simulink model "clutch_debug_simulink"  (R2024b)
settings: Solver=ode15s  StartTime=0.0  StopTime=4  MaxStep=0.002  RelTol=1e-6  AbsTol=1e-8
model workspace (MAT data in the model file):
  J_input = 0.00354192570756
  J_load = 2000
  M_debug = 100
  N_clutch = 230
  clutch1_profile = [0  0; 0.05  0; 0.06  0.1; 0.5  0.1; 0.7  1; 3  1; 3.1  0; 4  0]
  clutch2_profile = [0  0; 4  0]
  mi_c = 0.3
  mi_s = 0.4
  n_surfaces = 20
  r_eq_clutch = 0.1
  ratio1 = 3
  ratio2 = 1.5
  sigma0 = 335063
  sigma1 = 10
  sigma2 = 0
  vs = 0.5
libraries: simulink x6
settings Model: Creator=menda  LastModifiedBy=menda

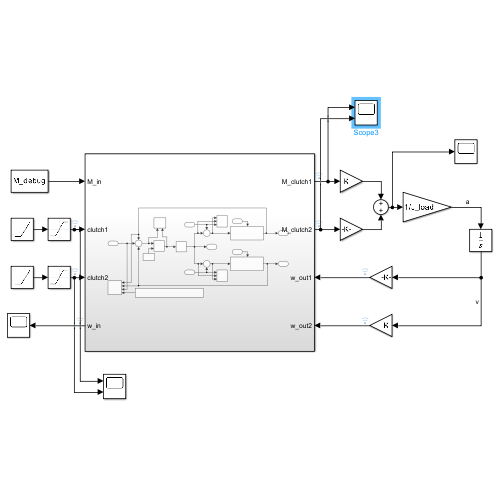
[thumbnail: Simulink's stored preview of the top-level diagram]
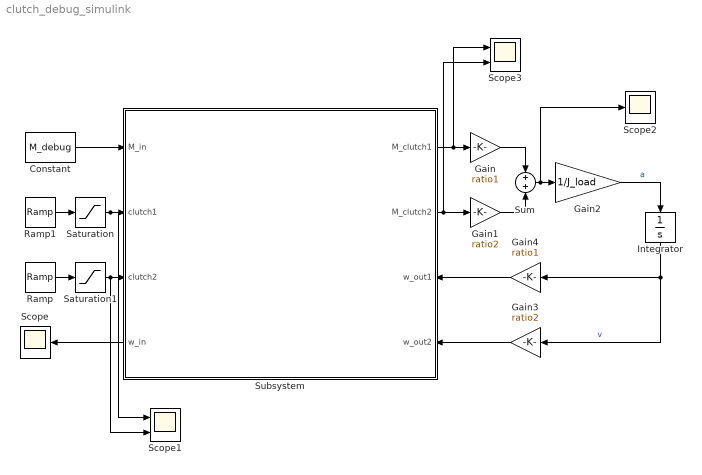
== system clutch_debug_simulink ==
  Constant : Constant  Value=M_debug
  Gain : Gain  Gain=ratio1
  Gain1 : Gain  Gain=ratio2
  Gain2 : Gain  Gain=1/J_load
  Gain3 : Gain  Gain=ratio2
  Gain4 : Gain  Gain=ratio1
  Integrator : Integrator  InitialCondition=100
  Ramp : simulink/Sources/Ramp  slope=3  start=1  InitialOutput=0
  Ramp1 : simulink/Sources/Ramp  slope=-3  start=1  InitialOutput=1
  Saturation : Saturate  UpperLimit=1  LowerLimit=0
  Saturation1 : Saturate  UpperLimit=1  LowerLimit=0
  Scope : Scope
  Scope1 : Scope  NumInputPorts=2
  Scope2 : Scope
  Scope3 : Scope  NumInputPorts=2
  Subsystem : Subsystem
      settings: PortSchema="{\"entries\":[{\"content\":{\"sides\":[{\"content\":{\"connectorIds\":[\"In1\",\"In2\",\"In3\",\"Out3\"]},\"type\":\"ConnectorPlacement.EquallySpacedRectSide\",\"uuid\":\"80fb4076-f99e-49a2-a4a4-074ad4e3703f\"},{\"content\":{\"connectorIds\":[\"Out1\",\"Out2\",\"In4\",\"In5\"],\"side\":\"RIGHT\"},\"type\":\"ConnectorPlacement.EquallySpacedRectSide\",\"uuid\":\"6fd981d1-b0c4-4e88-a9ee-be732220d23b\"},{\"content\":{\"side\":\"TOP\"},\"type\":\"ConnectorPlacement.EquallySpacedRectSide\",\"uuid\":\"d51b7d36-7666-4ef4-83a7-fb6ef995ec7f\"}]},\"type\":\"ConnectorPlacement.EquallySpacedConnector\",\"uuid\":\"9caa9749-ac4c-4898-95ff-5d55f9fdcdc9\"}],\"packageUris\":[\"http://schema.mathworks.com/mf0/Connector/R2020b\"],\"version\":\"1.0\"}"
  Sum : Sum  Inputs=+|+
  wires:
  Subsystem/1(M_clutch1) -> Scope3/1, Gain/1
  Subsystem/2(M_clutch2) -> Gain1/1, Scope3/2
  Constant/1 -> Subsystem/1(M_in)
  Saturation/1 -> Scope1/1, Subsystem/2(clutch1)
  Saturation1/1 -> Scope1/2, Subsystem/3(clutch2)
  Subsystem/3(w_in) -> Scope/1
  Gain/1 -> Sum/1
  Gain1/1 -> Sum/2
  Sum/1 -> Scope2/1, Gain2/1
  Gain2/1 -> Integrator/1  "a"
  Integrator/1 -> Gain3/1, Gain4/1  "v"
  Gain3/1 -> Subsystem/5(w_out2)
  Gain4/1 -> Subsystem/4(w_out1)
  Ramp1/1 -> Saturation/1
  Ramp/1 -> Saturation1/1

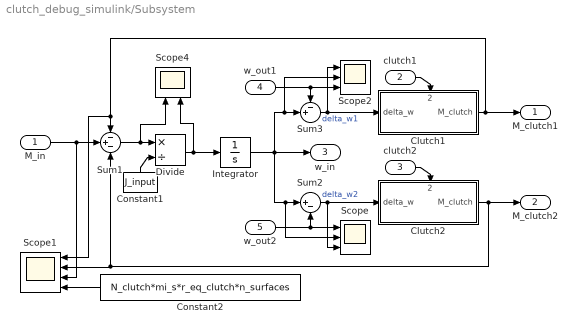
== system clutch_debug_simulink/Subsystem ==
  M_in : Inport
  clutch1 : Inport  Port=2
  clutch2 : Inport  Port=3
  w_out1 : Inport  Port=4
  w_out2 : Inport  Port=5
  Clutch1 : Subsystem
      settings: PortSchema="{\"entries\":[{\"content\":{\"sides\":[{\"content\":{\"connectorIds\":[\"In1\"]},\"type\":\"ConnectorPlacement.EquallySpacedRectSide\",\"uuid\":\"a26f5a32-9f9c-4306-b7a8-6355090a4a86\"},{\"content\":{\"connectorIds\":[\"Out1\"],\"side\":\"RIGHT\"},\"type\":\"ConnectorPlacement.EquallySpacedRectSide\",\"uuid\":\"4fa489e2-cd1d-4a36-b0cb-261100046200\"},{\"content\":{\"connectorIds\":[\"In2\"],\"side\":\"TOP\"},\"type\":\"ConnectorPlacement.EquallySpacedRectSide\",\"uuid\":\"0e05a540-d6e3-4351-9a32-83f6c32571ff\"}]},\"type\":\"ConnectorPlacement.EquallySpacedConnector\",\"uuid\":\"492e0439-728a-4999-b29b-e2639b0e762e\"}],\"packageUris\":[\"http://schema.mathworks.com/mf0/Connector/R2020b\"],\"version\":\"1.0\"}"
  Clutch2 : Subsystem
      settings: PortSchema="{\"entries\":[{\"content\":{\"sides\":[{\"content\":{\"connectorIds\":[\"In1\"]},\"type\":\"ConnectorPlacement.EquallySpacedRectSide\",\"uuid\":\"a26f5a32-9f9c-4306-b7a8-6355090a4a86\"},{\"content\":{\"connectorIds\":[\"Out1\"],\"side\":\"RIGHT\"},\"type\":\"ConnectorPlacement.EquallySpacedRectSide\",\"uuid\":\"4fa489e2-cd1d-4a36-b0cb-261100046200\"},{\"content\":{\"connectorIds\":[\"In2\"],\"side\":\"TOP\"},\"type\":\"ConnectorPlacement.EquallySpacedRectSide\",\"uuid\":\"0e05a540-d6e3-4351-9a32-83f6c32571ff\"}]},\"type\":\"ConnectorPlacement.EquallySpacedConnector\",\"uuid\":\"492e0439-728a-4999-b29b-e2639b0e762e\"}],\"packageUris\":[\"http://schema.mathworks.com/mf0/Connector/R2020b\"],\"version\":\"1.0\"}"
  Constant1 : Constant  Value=J_input
  Constant2 : Constant  Value=N_clutch*mi_s*r_eq_clutch*n_surfaces
  Divide : Product  Inputs=*/
  Integrator : Integrator  InitialCondition=100
  Scope : Scope  NumInputPorts=3
  Scope1 : Scope  NumInputPorts=4
  Scope2 : Scope  NumInputPorts=3
  Scope4 : Scope  NumInputPorts=2
  Sum1 : Sum  Inputs=-+-
  Sum2 : Sum  Inputs=|+-
  Sum3 : Sum  Inputs=-+|
  M_clutch1 : Outport
  M_clutch2 : Outport  Port=2
  w_in : Outport  Port=3
  wires:
  Sum3/1 -> Clutch1/1(delta_w), Scope2/1  "delta_w1"
  w_out1/1 -> Scope2/3, Sum3/1
  Clutch2/1(M_clutch) -> M_clutch2/1, Scope1/2, Sum1/3
  Sum1/1 -> Scope4/1, Divide/1
  Constant1/1 -> Divide/2
  w_out2/1 -> Scope/1, Sum2/2
  Integrator/1 -> w_in/1, Scope/2, Sum2/1, Scope2/2, Sum3/2
  Clutch1/1(M_clutch) -> M_clutch1/1, Scope1/1, Sum1/1
  clutch1/1 -> Clutch1/2(" ")
  Divide/1 -> Integrator/1, Scope4/2
  Constant2/1 -> Scope1/4
  Sum2/1 -> Clutch2/1(delta_w), Scope/3  "delta_w2"
  M_in/1 -> Sum1/2, Scope1/3
  clutch2/1 -> Clutch2/2(" ")

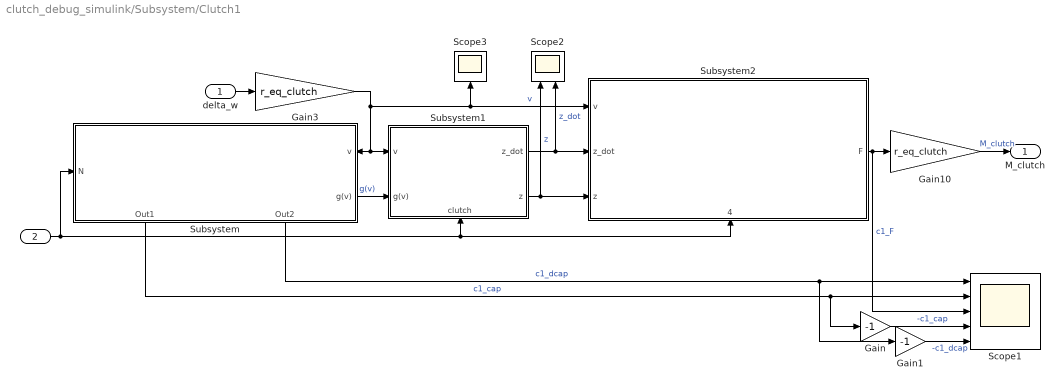
== system clutch_debug_simulink/Subsystem/Clutch1 ==
  delta_w : Inport
  " " : Inport  Port=2
  Gain : Gain  Gain=-1
  Gain1 : Gain  Gain=-1
  Gain10 : Gain  Gain=r_eq_clutch
  Gain3 : Gain  Gain=r_eq_clutch
  Scope1 : Scope  NumInputPorts=5
  Scope2 : Scope  NumInputPorts=2
  Scope3 : Scope
  Subsystem : Subsystem
      settings: PortSchema="{\"entries\":[{\"content\":{\"sides\":[{\"content\":{\"connectorIds\":[\"In1\"]},\"type\":\"ConnectorPlacement.EquallySpacedRectSide\",\"uuid\":\"0ae2ed28-5be6-4ce0-b87c-2c13a72d1ad0\"},{\"content\":{\"connectorIds\":[\"In2\",\"Out1\"],\"side\":\"RIGHT\"},\"type\":\"ConnectorPlacement.EquallySpacedRectSide\",\"uuid\":\"8d48d664-ebaf-4c3e-be9e-f793543e8061\"},{\"content\":{\"side\":\"TOP\"},\"type\":\"ConnectorPlacement.EquallySpacedRectSide\",\"uuid\":\"2d66836a-de46-4974-a48b-ee2778be1c08\"},{\"content\":{\"connectorIds\":[\"Out2\",\"Out3\"],\"side\":\"BOTTOM\"},\"type\":\"ConnectorPlacement.EquallySpacedRectSide\",\"uuid\":\"e232d9f4-6257-4976-8384-26c462ae0041\"}]},\"type\":\"ConnectorPlacement.EquallySpacedConnector\",\"uuid\":\"ae24f926-3a59-4a74-9cf0-af55dcfbad19\"}],\"packageUris\":[\"http://schema.mathworks.com/mf0/Connector/R2020b\"],\"version\":\"1.0\"}"
      mask Display: image('images/Stribeck.png');
  Subsystem1 : Subsystem
      settings: PortSchema="{\"entries\":[{\"content\":{\"sides\":[{\"content\":{\"connectorIds\":[\"In1\",\"In2\"]},\"type\":\"ConnectorPlacement.EquallySpacedRectSide\",\"uuid\":\"fba00446-fe01-4fd0-a740-7d5efbf0abc7\"},{\"content\":{\"connectorIds\":[\"Out1\",\"Out2\"],\"side\":\"RIGHT\"},\"type\":\"ConnectorPlacement.EquallySpacedRectSide\",\"uuid\":\"28d31996-59d3-4656-988b-c785e0d07c46\"},{\"content\":{\"side\":\"TOP\"},\"type\":\"ConnectorPlacement.EquallySpacedRectSide\",\"uuid\":\"07dfb693-bdac-419f-bf8c-22f11bb5a1ff\"},{\"content\":{\"connectorIds\":[\"In3\"],\"side\":\"BOTTOM\"},\"type\":\"ConnectorPlacement.EquallySpacedRectSide\",\"uuid\":\"e46b7f0d-22dc-4b01-9fc3-2183fe5bd14e\"}]},\"type\":\"ConnectorPlacement.EquallySpacedConnector\",\"uuid\":\"53afe5e8-6f41-4676-b5a4-a094561728b0\"}],\"packageUris\":[\"http://schema.mathworks.com/mf0/Connector/R2020b\"],\"version\":\"1.0\"}"
      mask Display: image('images/z_state.png');
  Subsystem2 : Subsystem
      settings: PortSchema="{\"entries\":[{\"content\":{\"sides\":[{\"content\":{\"connectorIds\":[\"In1\",\"In2\",\"In3\"]},\"type\":\"ConnectorPlacement.EquallySpacedRectSide\",\"uuid\":\"718e9a4c-012a-432e-af1d-56a8c510a1ff\"},{\"content\":{\"connectorIds\":[\"Out1\"],\"side\":\"RIGHT\"},\"type\":\"ConnectorPlacement.EquallySpacedRectSide\",\"uuid\":\"b8acef94-ef29-40e0-b6df-913e21cb4db2\"},{\"content\":{\"side\":\"TOP\"},\"type\":\"ConnectorPlacement.EquallySpacedRectSide\",\"uuid\":\"42ba6916-bf07-457b-89e7-b10a87e70d96\"},{\"content\":{\"connectorIds\":[\"In4\"],\"side\":\"BOTTOM\"},\"type\":\"ConnectorPlacement.EquallySpacedRectSide\",\"uuid\":\"25c3a005-357f-4967-9fb3-686ba180841f\"}]},\"type\":\"ConnectorPlacement.EquallySpacedConnector\",\"uuid\":\"db3b50fc-f4cd-400b-b8f7-b0301a8ba65b\"}],\"packageUris\":[\"http://schema.mathworks.com/mf0/Connector/R2020b\"],\"version\":\"1.0\"}"
      mask Display: image('images/fric_force.png');
  M_clutch : Outport
  wires:
  delta_w/1 -> Gain3/1
  Subsystem1/2(z) -> Scope2/1, Subsystem2/3(z)  "z"
  Subsystem1/1(z_dot) -> Scope2/2, Subsystem2/2(z_dot)  "z_dot"
  Subsystem2/1(F) -> Scope1/3, Gain10/1  "c1_F"
  Gain10/1 -> M_clutch/1  "M_clutch"
  Gain3/1 -> Scope3/1, Subsystem2/1(v), Subsystem1/1(v), Subsystem/2(v)  "v"
  Subsystem/1(g(v)) -> Subsystem1/2(g(v))  "g(v)"
  " "/1 -> Subsystem2/4(" "), Subsystem1/3("clutch "), Subsystem/1(N)
  Subsystem/2(Out1) -> Gain/1, Scope1/2  "c1_cap"
  Gain/1 -> Scope1/4  "-c1_cap"
  Subsystem/3(Out2) -> Gain1/1, Scope1/1  "c1_dcap"
  Gain1/1 -> Scope1/5  "-c1_dcap"

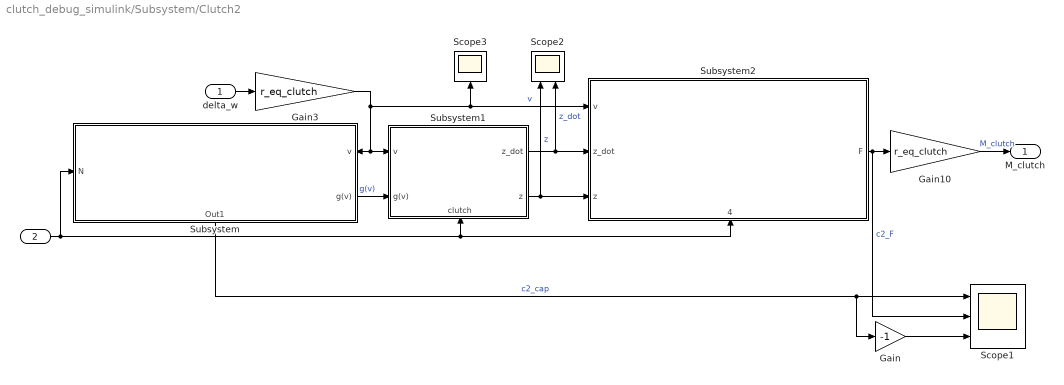
== system clutch_debug_simulink/Subsystem/Clutch2 ==
  delta_w : Inport
  " " : Inport  Port=2
  Gain : Gain  Gain=-1
  Gain10 : Gain  Gain=r_eq_clutch
  Gain3 : Gain  Gain=r_eq_clutch
  Scope1 : Scope  NumInputPorts=3
  Scope2 : Scope  NumInputPorts=2
  Scope3 : Scope
  Subsystem : Subsystem
      settings: PortSchema="{\"entries\":[{\"content\":{\"sides\":[{\"content\":{\"connectorIds\":[\"In1\"]},\"type\":\"ConnectorPlacement.EquallySpacedRectSide\",\"uuid\":\"0ae2ed28-5be6-4ce0-b87c-2c13a72d1ad0\"},{\"content\":{\"connectorIds\":[\"In2\",\"Out1\"],\"side\":\"RIGHT\"},\"type\":\"ConnectorPlacement.EquallySpacedRectSide\",\"uuid\":\"8d48d664-ebaf-4c3e-be9e-f793543e8061\"},{\"content\":{\"side\":\"TOP\"},\"type\":\"ConnectorPlacement.EquallySpacedRectSide\",\"uuid\":\"2d66836a-de46-4974-a48b-ee2778be1c08\"},{\"content\":{\"connectorIds\":[\"Out2\"],\"side\":\"BOTTOM\"},\"type\":\"ConnectorPlacement.EquallySpacedRectSide\",\"uuid\":\"e232d9f4-6257-4976-8384-26c462ae0041\"}]},\"type\":\"ConnectorPlacement.EquallySpacedConnector\",\"uuid\":\"ae24f926-3a59-4a74-9cf0-af55dcfbad19\"}],\"packageUris\":[\"http://schema.mathworks.com/mf0/Connector/R2020b\"],\"version\":\"1.0\"}"
      mask Display: image('images/Stribeck.png');
  Subsystem1 : Subsystem
      settings: PortSchema="{\"entries\":[{\"content\":{\"sides\":[{\"content\":{\"connectorIds\":[\"In1\",\"In2\"]},\"type\":\"ConnectorPlacement.EquallySpacedRectSide\",\"uuid\":\"fba00446-fe01-4fd0-a740-7d5efbf0abc7\"},{\"content\":{\"connectorIds\":[\"Out1\",\"Out2\"],\"side\":\"RIGHT\"},\"type\":\"ConnectorPlacement.EquallySpacedRectSide\",\"uuid\":\"28d31996-59d3-4656-988b-c785e0d07c46\"},{\"content\":{\"side\":\"TOP\"},\"type\":\"ConnectorPlacement.EquallySpacedRectSide\",\"uuid\":\"07dfb693-bdac-419f-bf8c-22f11bb5a1ff\"},{\"content\":{\"connectorIds\":[\"In3\"],\"side\":\"BOTTOM\"},\"type\":\"ConnectorPlacement.EquallySpacedRectSide\",\"uuid\":\"e46b7f0d-22dc-4b01-9fc3-2183fe5bd14e\"}]},\"type\":\"ConnectorPlacement.EquallySpacedConnector\",\"uuid\":\"53afe5e8-6f41-4676-b5a4-a094561728b0\"}],\"packageUris\":[\"http://schema.mathworks.com/mf0/Connector/R2020b\"],\"version\":\"1.0\"}"
      mask Display: image('images/z_state.png');
  Subsystem2 : Subsystem
      settings: PortSchema="{\"entries\":[{\"content\":{\"sides\":[{\"content\":{\"connectorIds\":[\"In1\",\"In2\",\"In3\"]},\"type\":\"ConnectorPlacement.EquallySpacedRectSide\",\"uuid\":\"718e9a4c-012a-432e-af1d-56a8c510a1ff\"},{\"content\":{\"connectorIds\":[\"Out1\"],\"side\":\"RIGHT\"},\"type\":\"ConnectorPlacement.EquallySpacedRectSide\",\"uuid\":\"b8acef94-ef29-40e0-b6df-913e21cb4db2\"},{\"content\":{\"side\":\"TOP\"},\"type\":\"ConnectorPlacement.EquallySpacedRectSide\",\"uuid\":\"42ba6916-bf07-457b-89e7-b10a87e70d96\"},{\"content\":{\"connectorIds\":[\"In4\"],\"side\":\"BOTTOM\"},\"type\":\"ConnectorPlacement.EquallySpacedRectSide\",\"uuid\":\"25c3a005-357f-4967-9fb3-686ba180841f\"}]},\"type\":\"ConnectorPlacement.EquallySpacedConnector\",\"uuid\":\"db3b50fc-f4cd-400b-b8f7-b0301a8ba65b\"}],\"packageUris\":[\"http://schema.mathworks.com/mf0/Connector/R2020b\"],\"version\":\"1.0\"}"
      mask Display: image('images/fric_force.png');
  M_clutch : Outport
  wires:
  Subsystem/2(Out1) -> Gain/1, Scope1/1  "c2_cap"
  " "/1 -> Subsystem/1(N), Subsystem1/3("clutch "), Subsystem2/4(" ")
  Subsystem/1(g(v)) -> Subsystem1/2(g(v))  "g(v)"
  Gain3/1 -> Subsystem/2(v), Subsystem1/1(v), Subsystem2/1(v), Scope3/1  "v"
  Gain10/1 -> M_clutch/1  "M_clutch"
  Subsystem2/1(F) -> Gain10/1, Scope1/2  "c2_F"
  Subsystem1/1(z_dot) -> Subsystem2/2(z_dot), Scope2/2  "z_dot"
  Subsystem1/2(z) -> Subsystem2/3(z), Scope2/1  "z"
  delta_w/1 -> Gain3/1
  Gain/1 -> Scope1/3

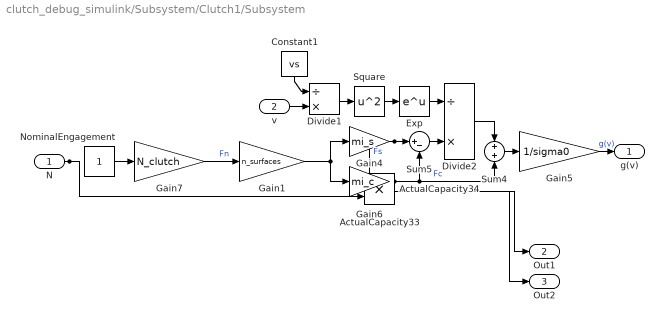
== system clutch_debug_simulink/Subsystem/Clutch1/Subsystem ==
  N : Inport
  v : Inport  Port=2
  ActualCapacity33 : Product
  ActualCapacity34 : Product
  Constant1 : Constant  Value=vs
  Divide1 : Product  Inputs=/*
  Divide2 : Product  Inputs=/*
  Exp : Math
  Gain1 : Gain  Gain=n_surfaces
  Gain4 : Gain  Gain=mi_s
  Gain5 : Gain  Gain=1/sigma0
  Gain6 : Gain  Gain=mi_c
  Gain7 : Gain  Gain=N_clutch
  NominalEngagement : Constant
  Square : Math  Operator=square
  Sum4 : Sum  Inputs=+|+
  Sum5 : Sum  Inputs=|+-
  g(v) : Outport
  Out1 : Outport  Port=2
  Out2 : Outport  Port=3
  wires:
  Gain1/1 -> Gain4/1, Gain6/1
  Gain4/1 -> Sum5/1, ActualCapacity33/1  "Fs"
  v/1 -> Divide1/2
  N/1 -> ActualCapacity33/2, ActualCapacity34/2
  Gain5/1 -> g(v)/1  "g(v)"
  Square/1 -> Exp/1
  Divide1/1 -> Square/1
  Constant1/1 -> Divide1/1
  Gain7/1 -> Gain1/1  "Fn"
  Exp/1 -> Divide2/1
  Gain6/1 -> Sum5/2, Sum4/2, ActualCapacity34/1  "Fc"
  Divide2/1 -> Sum4/1
  Sum5/1 -> Divide2/2
  Sum4/1 -> Gain5/1
  NominalEngagement/1 -> Gain7/1
  ActualCapacity33/1 -> Out1/1
  ActualCapacity34/1 -> Out2/1

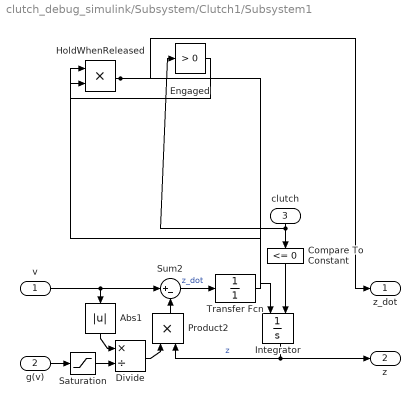
== system clutch_debug_simulink/Subsystem/Clutch1/Subsystem1 ==
  v : Inport
  g(v) : Inport  Port=2
  "clutch " : Inport  Port=3
  Abs1 : Abs  SaturateOnIntegerOverflow=off
  Compare To Constant : simulink/Logic and Bit Operations/Compare To Constant  relop=<=  const=0  OutDataTypeStr=boolean
  Divide : Product  Inputs=*/
  Engaged : simulink/Logic and Bit Operations/Compare To Constant  relop=>  const=0  OutDataTypeStr=boolean
  HoldWhenReleased : Product
  Integrator : Integrator  ExternalReset=rising
  Product2 : Product
  Saturation : Saturate  UpperLimit=inf  LowerLimit=1e-12
  Sum2 : Sum  Inputs=|+-
  Transfer Fcn : TransferFcn  Numerator=1  Denominator=1
  z_dot : Outport
  z : Outport  Port=2
  wires:
  Compare To Constant/1 -> Integrator/2
  g(v)/1 -> Saturation/1
  Product2/1 -> Sum2/2
  Abs1/1 -> Divide/1
  Saturation/1 -> Divide/2
  Sum2/1 -> Transfer Fcn/1  "z_dot"
  v/1 -> Sum2/1, Abs1/1
  Divide/1 -> Product2/1
  Integrator/1 -> z/1, Product2/2  "z"
  "clutch "/1 -> Compare To Constant/1, Engaged/1
  Transfer Fcn/1 -> HoldWhenReleased/1
  Engaged/1 -> HoldWhenReleased/2
  HoldWhenReleased/1 -> z_dot/1, Integrator/1

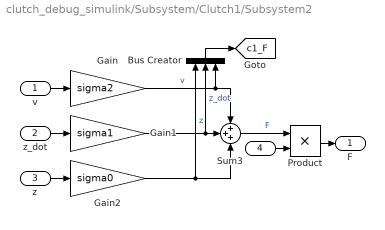
== system clutch_debug_simulink/Subsystem/Clutch1/Subsystem2 ==
  v : Inport
  z_dot : Inport  Port=2
  z : Inport  Port=3
  " " : Inport  Port=4
  Bus Creator : BusCreator  Inputs=3
  Gain : Gain  Gain=sigma2
  Gain1 : Gain  Gain=sigma1
  Gain2 : Gain  Gain=sigma0
  Product : Product
  Sum3 : Sum  Inputs=+++
  F : Outport
  tag scope: c1_F=global
  wires:
  z/1 -> Gain2/1
  z_dot/1 -> Gain1/1
  Gain1/1 -> Bus Creator/2, Sum3/2  "z_dot"
  Sum3/1 -> Product/1  "F"
  Gain2/1 -> Bus Creator/1, Sum3/3  "z"
  Gain/1 -> Bus Creator/3, Sum3/1  "v"
  v/1 -> Gain/1
  " "/1 -> Product/2
  Product/1 -> F/1
  Bus Creator/1 -> [c1_F]

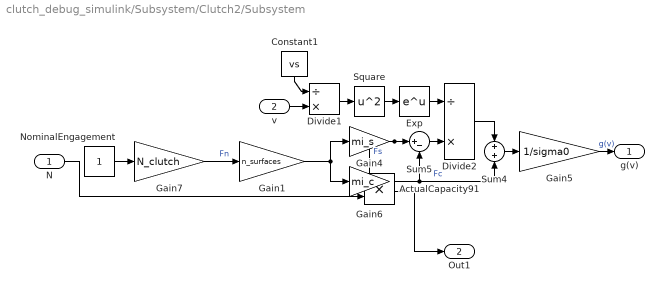
== system clutch_debug_simulink/Subsystem/Clutch2/Subsystem ==
  N : Inport
  v : Inport  Port=2
  ActualCapacity91 : Product
  Constant1 : Constant  Value=vs
  Divide1 : Product  Inputs=/*
  Divide2 : Product  Inputs=/*
  Exp : Math
  Gain1 : Gain  Gain=n_surfaces
  Gain4 : Gain  Gain=mi_s
  Gain5 : Gain  Gain=1/sigma0
  Gain6 : Gain  Gain=mi_c
  Gain7 : Gain  Gain=N_clutch
  NominalEngagement : Constant
  Square : Math  Operator=square
  Sum4 : Sum  Inputs=+|+
  Sum5 : Sum  Inputs=|+-
  g(v) : Outport
  Out1 : Outport  Port=2
  wires:
  Sum4/1 -> Gain5/1
  Sum5/1 -> Divide2/2
  Divide2/1 -> Sum4/1
  Gain6/1 -> Sum4/2, Sum5/2  "Fc"
  Exp/1 -> Divide2/1
  Gain7/1 -> Gain1/1  "Fn"
  Constant1/1 -> Divide1/1
  Divide1/1 -> Square/1
  Square/1 -> Exp/1
  Gain5/1 -> g(v)/1  "g(v)"
  N/1 -> ActualCapacity91/2
  v/1 -> Divide1/2
  Gain4/1 -> Sum5/1, ActualCapacity91/1  "Fs"
  Gain1/1 -> Gain6/1, Gain4/1
  NominalEngagement/1 -> Gain7/1
  ActualCapacity91/1 -> Out1/1

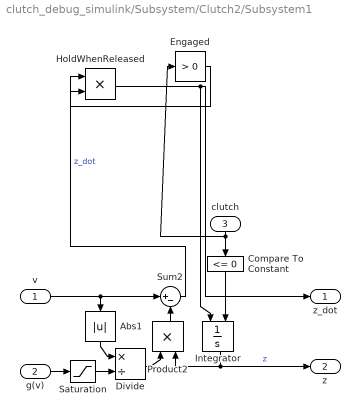
== system clutch_debug_simulink/Subsystem/Clutch2/Subsystem1 ==
  v : Inport
  g(v) : Inport  Port=2
  "clutch " : Inport  Port=3
  Abs1 : Abs  SaturateOnIntegerOverflow=off
  Compare To Constant : simulink/Logic and Bit Operations/Compare To Constant  relop=<=  const=0  OutDataTypeStr=boolean
  Divide : Product  Inputs=*/
  Engaged : simulink/Logic and Bit Operations/Compare To Constant  relop=>  const=0  OutDataTypeStr=boolean
  HoldWhenReleased : Product
  Integrator : Integrator  ExternalReset=rising
  Product2 : Product
  Saturation : Saturate  UpperLimit=inf  LowerLimit=1e-12
  Sum2 : Sum  Inputs=|+-
  z_dot : Outport
  z : Outport  Port=2
  wires:
  "clutch "/1 -> Compare To Constant/1, Engaged/1
  Integrator/1 -> Product2/2, z/1  "z"
  Divide/1 -> Product2/1
  v/1 -> Abs1/1, Sum2/1
  Saturation/1 -> Divide/2
  Abs1/1 -> Divide/1
  Product2/1 -> Sum2/2
  g(v)/1 -> Saturation/1
  Compare To Constant/1 -> Integrator/2
  Sum2/1 -> HoldWhenReleased/1  "z_dot"
  Engaged/1 -> HoldWhenReleased/2
  HoldWhenReleased/1 -> Integrator/1, z_dot/1

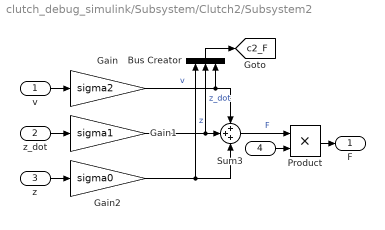
== system clutch_debug_simulink/Subsystem/Clutch2/Subsystem2 ==
  v : Inport
  z_dot : Inport  Port=2
  z : Inport  Port=3
  " " : Inport  Port=4
  Bus Creator : BusCreator  Inputs=3
  Gain : Gain  Gain=sigma2
  Gain1 : Gain  Gain=sigma1
  Gain2 : Gain  Gain=sigma0
  Product : Product
  Sum3 : Sum  Inputs=+++
  F : Outport
  tag scope: c2_F=global
  wires:
  Bus Creator/1 -> [c2_F]
  Product/1 -> F/1
  " "/1 -> Product/2
  v/1 -> Gain/1
  Gain/1 -> Sum3/1, Bus Creator/3  "v"
  Gain2/1 -> Sum3/3, Bus Creator/1  "z"
  Sum3/1 -> Product/1  "F"
  Gain1/1 -> Sum3/2, Bus Creator/2  "z_dot"
  z_dot/1 -> Gain1/1
  z/1 -> Gain2/1
